simulink model "srmc_controller"  (R2025a)
settings: Solver=ode3  StartTime=0.0  StopTime=86400  FixedStep=5  RelTol=1e-3
undefined symbols (not defined in the file): sched_angles, sched_hours
libraries: simulink x3
settings Model: Creator=ELCOT  LastModifiedBy=ELCOT

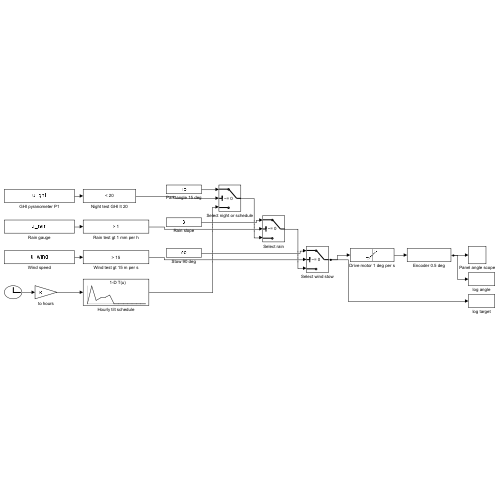
[thumbnail: Simulink's stored preview of the top-level diagram]
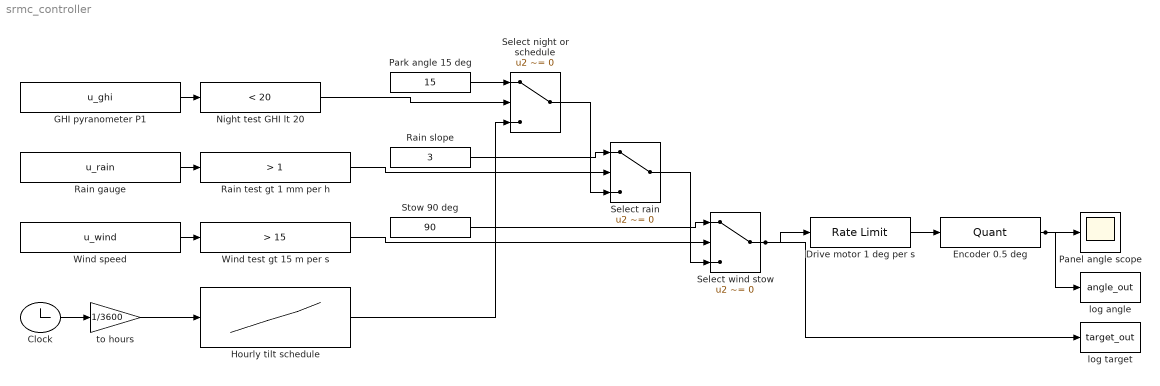
== system srmc_controller ==
  Clock : Clock
  Drive motor 1 deg per s : RateLimiter  SampleTimeMode=inherited
  Encoder 0.5 deg : Quantizer
  GHI pyranometer P1 : FromWorkspace  VariableName=u_ghi
  Hourly tilt schedule : Lookup_n-D  NumberOfTableDimensions=1  BreakpointsForDimension1=sched_hours  Table=sched_angles  ExtrapMethod=Clip  InternalRulePriority=Speed  RndMeth=Simplest
  Night test GHI lt 20 : simulink/Logic and Bit Operations/Compare To Constant  relop=<  const=20  OutDataTypeStr=boolean
  Panel angle scope : Scope
  Park angle 15 deg : Constant  Value=15
  Rain gauge : FromWorkspace  VariableName=u_rain
  Rain slope : Constant  Value=3
  Rain test gt 1 mm per h : simulink/Logic and Bit Operations/Compare To Constant  relop=>  const=1  OutDataTypeStr=boolean
  Select night or schedule : Switch  Criteria=u2 ~= 0  SaturateOnIntegerOverflow=off  InputSameDT=off
  Select rain : Switch  Criteria=u2 ~= 0  SaturateOnIntegerOverflow=off  InputSameDT=off
  Select wind stow : Switch  Criteria=u2 ~= 0  SaturateOnIntegerOverflow=off  InputSameDT=off
  Stow 90 deg : Constant  Value=90
  Wind speed : FromWorkspace  VariableName=u_wind
  Wind test gt 15 m per s : simulink/Logic and Bit Operations/Compare To Constant  relop=>  const=15  OutDataTypeStr=boolean
  log angle : ToWorkspace  VariableName=angle_out  SaveFormat=Timeseries  SampleTime=-1
  log target : ToWorkspace  VariableName=target_out  SaveFormat=Timeseries  SampleTime=-1
  to hours : Gain  Gain=1/3600
  wires:
  GHI pyranometer P1/1 -> Night test GHI lt 20/1
  Rain gauge/1 -> Rain test gt 1 mm per h/1
  Wind speed/1 -> Wind test gt 15 m per s/1
  Clock/1 -> to hours/1
  to hours/1 -> Hourly tilt schedule/1
  Park angle 15 deg/1 -> Select night or schedule/1
  Night test GHI lt 20/1 -> Select night or schedule/2
  Hourly tilt schedule/1 -> Select night or schedule/3
  Rain slope/1 -> Select rain/1
  Rain test gt 1 mm per h/1 -> Select rain/2
  Select night or schedule/1 -> Select rain/3
  Stow 90 deg/1 -> Select wind stow/1
  Wind test gt 15 m per s/1 -> Select wind stow/2
  Select rain/1 -> Select wind stow/3
  Select wind stow/1 -> Drive motor 1 deg per s/1, log target/1
  Drive motor 1 deg per s/1 -> Encoder 0.5 deg/1
  Encoder 0.5 deg/1 -> Panel angle scope/1, log angle/1
